simulink model "untitled"  (R2018a)
settings: Solver=VariableStepAuto  StartTime=0.0  StopTime=6.0  RelTol=1e-3
undefined symbols (not defined in the file or in its folder): b2, n2, nazivnik2
settings Model: Creator=janko  LastModifiedBy=janko

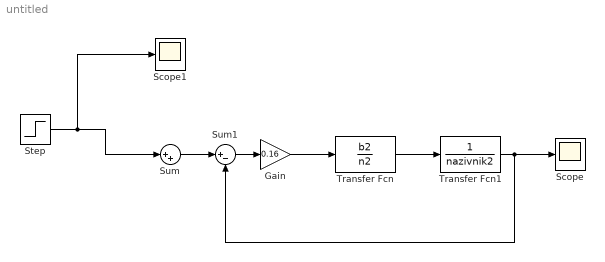
== system untitled ==
  Gain : Gain  Gain=0.16
  Scope : Scope
  Scope1 : Scope
  Step : Step  After=10  SampleTime=0
  Sum : Sum  Inputs=|++
  Sum1 : Sum  Inputs=|+-
  Transfer Fcn : TransferFcn  Numerator=b2  Denominator=n2
  Transfer Fcn1 : TransferFcn  Numerator=1  Denominator=nazivnik2
  wires:
  Step/1 -> Scope1/1, Sum/1
  Sum/1 -> Sum1/1
  Gain/1 -> Transfer Fcn/1
  Sum1/1 -> Gain/1
  Transfer Fcn/1 -> Transfer Fcn1/1
  Transfer Fcn1/1 -> Scope/1, Sum1/2
